simulink model "ellipsoidSMC"  (R2024a)
settings: Solver=ode45  StartTime=0  StopTime=350  FixedStep=0.01  MaxStep=0.01  RelTol=1e-4  AbsTol=1e-4  EnableMultiTasking=on
values from neighbouring files (symbols this model uses):
  simu = simulationClass()    [wecSimInputFile.m]
  waves = waveClass('regular')    [wecSimInputFile.m]
undefined symbols (not defined in the file or in its folder): body, controller, pto, X, Y, Z
libraries: nesl_utility x22, sm_lib x16, WECSim_Lib_Body_Elements x6, WECSim_Lib_Frames x1, vrlib x1, WECSim_Lib_PTOs x1
(part 2 of 3)

== system ellipsoidSMC/Rigid Body/Hydrodynamic Body/Structure ==
  note: Apply the total force to the body and calculate its response relative to the global reference frame.
      |
      | Output force to apply to another body.
  Total Force : Inport
  Body Properties : sm_lib/Body Elements/File Solid  ExtGeomFileName=geometry/elipsoid.stl  UnitType=Custom  ExtGeomFileUnits=m  StepReaderType=HEX  ExportConvexHullGeometry=off  InertiaType=Custom  BasedOnType=Density  Density=1000  DensityUnits=kg/(m^3)  Mass=body.mass  MassUnits=kg  CenterOfMass=[0 0 0]  CenterOfMassUnits=m  MomentsOfInertia=body.inertia  MomentsOfInertiaUnits=kg*m^2  ProductsOfInertia=body.inertiaProducts  ProductsOfInertiaUnits=kg*m^2  GraphicType=FromGeometry  MarkerShape=Sphere  MarkerSize=10  GraphicVisPropType=SimpleVisualProperties  GraphicDiffuseColor=body.viz.color  GraphicOpacity=body.viz.opacity  GraphicSpecularColor=[0.5 0.5 0.5 1.0]  GraphicAmbientColor=[0.15 0.15 0.15 1.0]  GraphicEmissiveColor=[0.0 0.0 0.0 1.0]  GraphicShininess=75  DoExposeReferenceFrame=on  SerializedFrames=<Frames/>
  External Force and Torque : sm_lib/Forces and Torques/External Force and Torque  EnableForceX=off  EnableForceY=off  EnableForceZ=off  EnableForce=on  ForceResolutionFrame=World  EnableTorqueX=off  EnableTorqueY=off  EnableTorqueZ=off  EnableTorque=on  TorqueResolutionFrame=World
  Motion Sensor : Subsystem
  Rigid Transform (Setup CG) : sm_lib/Frames and Transforms/Rigid Transform  RotationMethod=None  FollAlignAxisA=+X  BaseAlignAxisA=+Y  FollAlignAxisB=+Y  BaseAlignAxisB=+Z  RotationStandardAxis=+Y  RotationAngle=0.05  RotationAngleUnits=rad  RotationArbitraryAxis=[0.57735026918962584 0.57735026918962584 0.57735026918962584]  RotationSequenceAxes=FollowerAxes  RotationSequence=XYX  RotationSequenceAngles=[0 0 0]  RotationSequenceAnglesUnits=deg  RotationMatrix=[1 0 0; 0 1 0; 0 0 1]  Quaternion=[1 0 0 0]  TranslationMethod=Cartesian  TranslationCartesianOffset=body.centerGravity  TranslationCartesianOffsetUnits=m  TranslationStandardAxis=+Z  TranslationStandardOffset=0  TranslationStandardOffsetUnits=m  TranslationROffset=0  TranslationROffsetUnits=m  TranslationThetaOffset=0  TranslationThetaOffsetUnits=deg  TranslationZOffset=0  TranslationZOffsetUnits=m
  Rigid Transform (Setup Initial Disp) : sm_lib/Frames and Transforms/Rigid Transform  RotationMethod=ArbitraryAxis  FollAlignAxisA=+X  BaseAlignAxisA=+Y  FollAlignAxisB=+Y  BaseAlignAxisB=+Z  RotationStandardAxis=+Y  RotationAngle=body.initial.angle  RotationAngleUnits=rad  RotationArbitraryAxis=body.initial.axis  RotationSequenceAxes=FollowerAxes  RotationSequence=XYX  RotationSequenceAngles=[0 0 0]  RotationSequenceAnglesUnits=deg  RotationMatrix=[1 0 0; 0 1 0; 0 0 1]  Quaternion=[1 0 0 0]  TranslationMethod=Cartesian  TranslationCartesianOffset=body.initial.displacement  TranslationCartesianOffsetUnits=m  TranslationStandardAxis=+Z  TranslationStandardOffset=0  TranslationStandardOffsetUnits=m  TranslationROffset=0  TranslationROffsetUnits=m  TranslationThetaOffset=0  TranslationThetaOffsetUnits=deg  TranslationZOffset=0  TranslationZOffsetUnits=m
  Selector : Selector  InputPortWidth=6  IndexOptions=Index vector (dialog)  Indices=[1:3]  OutputSizes=1
  Selector1 : Selector  InputPortWidth=6  IndexOptions=Index vector (dialog)  Indices=[4:6]  OutputSizes=1
  Simulink-PS Converter1 : nesl_utility/Simulink-PS Converter  PhysicalDomain=network_engine_domain  SubClassName=ps_input  LeftPortType=input  RightPortType=output  PseudoPeriodic=off  Frequencies=[]  NoiseDistribution=none  NoiseParameters=[]  Unit=1  AffineConversion=off  FilteringAndDerivatives=zero  SimscapeFilterOrder=1  InputFilterTimeConstant=0.001  UdotUserProvided=1
  Simulink-PS Converter2 : nesl_utility/Simulink-PS Converter  PhysicalDomain=network_engine_domain  SubClassName=ps_input  LeftPortType=input  RightPortType=output  PseudoPeriodic=off  Frequencies=[]  NoiseDistribution=none  NoiseParameters=[]  Unit=1  AffineConversion=off  FilteringAndDerivatives=zero  SimscapeFilterOrder=1  InputFilterTimeConstant=0.001  UdotUserProvided=1
  World Frame : sm_lib/Frames and Transforms/World Frame
  Conn Free Surface : PMIOPort  Side=Right
  Response : Outport
  wires:
  Total Force/1 -> Selector1/1, Selector/1
  Selector/1 -> Simulink-PS Converter1/1
  Selector1/1 -> Simulink-PS Converter2/1
  Motion Sensor/1(Response) -> Response/1
  connections:
  External Force and Torque/LConn1 -- Simulink-PS Converter1/RConn1
  External Force and Torque/LConn2 -- Simulink-PS Converter2/RConn1
  Rigid Transform (Setup Initial Disp)/RConn1 -- Body Properties/RConn1 -- External Force and Torque/RConn1 -- Motion Sensor/RConn1
  Conn Free Surface/RConn1 -- Rigid Transform (Setup CG)/LConn1
  Rigid Transform (Setup Initial Disp)/LConn1 -- Rigid Transform (Setup CG)/RConn1
  World Frame/RConn1 -- Motion Sensor/LConn1

== system ellipsoidSMC/Rigid Body/Hydrodynamic Body/Wave Diffraction and Excitation Force Calculation ==
  note: The excitation force = F_wave * ramp function
  Time : Inport
  Displacement : Inport  Port=2
  WaveElv : Inport  Port=3
  Add : Sum
  Constant : Constant
  FexcInputs : Subsystem
  Less Than : RelationalOperator  Operator=<  OutDataTypeStr=boolean  RndMeth=Simplest  InputSameDT=off
  Linear Wave Excitation Force Variant Subsystem : Subsystem  Variant=on  VariantControl=sv_irregularWavesNonLinYaw_b1  mask{Nwave=waves(1)}
      mask prompts: Nwave "Wave Instance"
  Nonlinear FK Force Variant Subsystem : Subsystem  Variant=on
  Product : Product
  Ramp Function Time : Constant  Value=simu.rampTime
  Ramp function : Subsystem
  Switch : Switch  Criteria=u2 ~= 0  SaturateOnIntegerOverflow=off  InputSameDT=off
  F_Excitation : Outport  PortDimensions=body.dof
  wires:
  FexcInputs/3(Out3) -> Nonlinear FK Force Variant Subsystem/3(WaveElv)
  WaveElv/1 -> FexcInputs/3(WaveElv)
  Displacement/1 -> FexcInputs/2(Displacement)
  Time/1 -> FexcInputs/1(Time)
  FexcInputs/1(Out1) -> Nonlinear FK Force Variant Subsystem/1(Time), Linear Wave Excitation Force Variant Subsystem/1(Time), Ramp function/1(Time), Less Than/1
  FexcInputs/2(Out2) -> Nonlinear FK Force Variant Subsystem/2(Displacement), Linear Wave Excitation Force Variant Subsystem/2(Displacement)
  Constant/1 -> Switch/3
  Less Than/1 -> Switch/2
  Ramp function/1(R) -> Switch/1
  Ramp Function Time/1 -> Less Than/2
  Nonlinear FK Force Variant Subsystem/1(Nonlinear Excitation) -> Add/2
  Linear Wave Excitation Force Variant Subsystem/1(Linear Excitation) -> Add/1
  Product/1 -> F_Excitation/1  "F_Excitation"
  Add/1 -> Product/2  "F_wave"
  Switch/1 -> Product/1  "R"

== system ellipsoidSMC/Rigid Body/Hydrodynamic Body/Wave Radiation Forces Calculation ==
  note: F_AddedMass = AM * a
  Velocity : Inport
  Acceleration : Inport  Port=2
  Added Mass Matrix : Constant  Value=body.hydroForce.fAddedMass
  Product1 : Product  Multiplication=Matrix(*)
  SS CI and Constant-Damping-CoeVariant Subsystem : Subsystem  Variant=on
  F_RadiationDamping : Outport
  F_AddedMass : Outport  Port=2
  wires:
  Acceleration/1 -> Product1/2
  SS CI and Constant-Damping-CoeVariant Subsystem/1(Out1) -> F_RadiationDamping/1  "F_RadiationDamping"
  Velocity/1 -> SS CI and Constant-Damping-CoeVariant Subsystem/1(velocity)
  Product1/1 -> F_AddedMass/1  "F_AddedMass"
  Added Mass Matrix/1 -> Product1/1

== system ellipsoidSMC/Rigid Body/Hydrodynamic Body/Yaw Force Transforms ==
  F_Excitation : Inport
  F_RadiationDamping : Inport  Port=2
  In2 : Inport  Port=3
  F_AddedMass : Inport  Port=4
  F_Restoring : Inport  Port=5
  Constant : Constant  Value=body.yaw.option
  Yaw Force Transforms : MATLAB Function  TreatAsAtomicUnit=on
  Out1 : Outport
  Out2 : Outport  Port=2
  Out3 : Outport  Port=3
  Out4 : Outport  Port=4
  wires:
  Yaw Force Transforms/1(F_Excitation) -> Out1/1
  Yaw Force Transforms/3(F_AddedMass) -> Out3/1
  Yaw Force Transforms/2(F_RadiationDamping) -> Out2/1
  F_RadiationDamping/1 -> Yaw Force Transforms/2(dispGlobal)
  F_AddedMass/1 -> Yaw Force Transforms/4(F_AddedMassLocal)
  Yaw Force Transforms/4(F_Restoring) -> Out4/1
  F_Excitation/1 -> Yaw Force Transforms/5(F_ExcitationLocal)
  In2/1 -> Yaw Force Transforms/3(F_RadiationDampingLocal)
  F_Restoring/1 -> Yaw Force Transforms/6(F_RestoringLocal)
  Constant/1 -> Yaw Force Transforms/1(yaw)

== system ellipsoidSMC/Rigid Body/Hydrodynamic Body/Yaw Kinematic Transforms ==
  note: If simu.b2b == 0, no body to body interaction is used (noB2B)
      | If simu.b2b == 1, use body to body interaction (B2B)
  note: 1) Add Subsystem or Model blocks as valid variant choices.
      | 2) You cannot connect blocks at this level. At simulation, connectivity is automatically
      | determined, based on the active variant and port name matching.
  dispGlobal : Inport
  velGlobal : Inport  Port=2
  accGlobal : Inport  Port=3
  No B2B : Subsystem  VariantControl=sv_noB2B
  With B2B : Subsystem  VariantControl=sv_B2B
  dispLoc : Outport
  velLoc : Outport  Port=2
  accLoc : Outport  Port=3

== system ellipsoidSMC/Rigid Body/Non-Hydro Body/Structure ==
  note: Apply the total force to the body and calculate its response relative to the global reference frame.
      |
      | Output force to apply to another body.
  Total Force : Inport
  Body Properties : sm_lib/Body Elements/File Solid  ExtGeomFileName=geometry/elipsoid.stl  UnitType=Custom  ExtGeomFileUnits=m  StepReaderType=HEX  ExportConvexHullGeometry=off  InertiaType=Custom  BasedOnType=Density  Density=1000  DensityUnits=kg/(m^3)  Mass=body.mass  MassUnits=kg  CenterOfMass=[0 0 0]  CenterOfMassUnits=m  MomentsOfInertia=body.inertia  MomentsOfInertiaUnits=kg*m^2  ProductsOfInertia=body.inertiaProducts  ProductsOfInertiaUnits=kg*m^2  GraphicType=FromGeometry  MarkerShape=Sphere  MarkerSize=10  GraphicVisPropType=SimpleVisualProperties  GraphicDiffuseColor=body.viz.color  GraphicOpacity=body.viz.opacity  GraphicSpecularColor=[0.5 0.5 0.5 1.0]  GraphicAmbientColor=[0.15 0.15 0.15 1.0]  GraphicEmissiveColor=[0.0 0.0 0.0 1.0]  GraphicShininess=75  DoExposeReferenceFrame=on  SerializedFrames=<Frames/>
  External Force and Torque : sm_lib/Forces and Torques/External Force and Torque  EnableForceX=off  EnableForceY=off  EnableForceZ=off  EnableForce=on  ForceResolutionFrame=World  EnableTorqueX=off  EnableTorqueY=off  EnableTorqueZ=off  EnableTorque=on  TorqueResolutionFrame=World
  Motion Sensor : WECSim_Lib_Body_Elements/Rigid Body/Hydrodynamic Body/Structure/Motion Sensor  SystemSampleTime=-1  VariantActivationTime=update diagram  AllowFlexibleInterface=on  Latency=0  AutoFrameSizeCalculation=off
  Rigid Transform (Setup CG) : sm_lib/Frames and Transforms/Rigid Transform  RotationMethod=None  FollAlignAxisA=+X  BaseAlignAxisA=+Y  FollAlignAxisB=+Y  BaseAlignAxisB=+Z  RotationStandardAxis=+Y  RotationAngle=0.05  RotationAngleUnits=rad  RotationArbitraryAxis=[0.57735026918962584 0.57735026918962584 0.57735026918962584]  RotationSequenceAxes=FollowerAxes  RotationSequence=XYX  RotationSequenceAngles=[0 0 0]  RotationSequenceAnglesUnits=deg  RotationMatrix=[1 0 0; 0 1 0; 0 0 1]  Quaternion=[1 0 0 0]  TranslationMethod=Cartesian  TranslationCartesianOffset=body.centerGravity  TranslationCartesianOffsetUnits=m  TranslationStandardAxis=+Z  TranslationStandardOffset=0  TranslationStandardOffsetUnits=m  TranslationROffset=0  TranslationROffsetUnits=m  TranslationThetaOffset=0  TranslationThetaOffsetUnits=deg  TranslationZOffset=0  TranslationZOffsetUnits=m
  Rigid Transform (Setup Initial Disp) : sm_lib/Frames and Transforms/Rigid Transform  RotationMethod=ArbitraryAxis  FollAlignAxisA=+X  BaseAlignAxisA=+Y  FollAlignAxisB=+Y  BaseAlignAxisB=+Z  RotationStandardAxis=+Y  RotationAngle=body.initial.angle  RotationAngleUnits=rad  RotationArbitraryAxis=body.initial.axis  RotationSequenceAxes=FollowerAxes  RotationSequence=XYX  RotationSequenceAngles=[0 0 0]  RotationSequenceAnglesUnits=deg  RotationMatrix=[1 0 0; 0 1 0; 0 0 1]  Quaternion=[1 0 0 0]  TranslationMethod=Cartesian  TranslationCartesianOffset=body.initial.displacement  TranslationCartesianOffsetUnits=m  TranslationStandardAxis=+Z  TranslationStandardOffset=0  TranslationStandardOffsetUnits=m  TranslationROffset=0  TranslationROffsetUnits=m  TranslationThetaOffset=0  TranslationThetaOffsetUnits=deg  TranslationZOffset=0  TranslationZOffsetUnits=m
  Selector : Selector  InputPortWidth=6  IndexOptions=Index vector (dialog)  Indices=[1:3]  OutputSizes=1
  Selector1 : Selector  InputPortWidth=6  IndexOptions=Index vector (dialog)  Indices=[4:6]  OutputSizes=1
  Simulink-PS Converter1 : nesl_utility/Simulink-PS Converter  PhysicalDomain=network_engine_domain  SubClassName=ps_input  LeftPortType=input  RightPortType=output  PseudoPeriodic=off  Frequencies=[]  NoiseDistribution=none  NoiseParameters=[]  Unit=1  AffineConversion=off  FilteringAndDerivatives=zero  SimscapeFilterOrder=1  InputFilterTimeConstant=0.001  UdotUserProvided=1
  Simulink-PS Converter2 : nesl_utility/Simulink-PS Converter  PhysicalDomain=network_engine_domain  SubClassName=ps_input  LeftPortType=input  RightPortType=output  PseudoPeriodic=off  Frequencies=[]  NoiseDistribution=none  NoiseParameters=[]  Unit=1  AffineConversion=off  FilteringAndDerivatives=zero  SimscapeFilterOrder=1  InputFilterTimeConstant=0.001  UdotUserProvided=1
  World Frame : sm_lib/Frames and Transforms/World Frame
  Conn Free Surface : PMIOPort  Side=Right
  Response : Outport
  wires:
  Total Force/1 -> Selector1/1, Selector/1
  Selector/1 -> Simulink-PS Converter1/1
  Selector1/1 -> Simulink-PS Converter2/1
  Motion Sensor/1 -> Response/1
  connections:
  External Force and Torque/LConn1 -- Simulink-PS Converter1/RConn1
  External Force and Torque/LConn2 -- Simulink-PS Converter2/RConn1
  Motion Sensor/RConn1 -- Body Properties/RConn1 -- Rigid Transform (Setup Initial Disp)/RConn1 -- External Force and Torque/RConn1
  Conn Free Surface/RConn1 -- Rigid Transform (Setup CG)/LConn1
  Rigid Transform (Setup Initial Disp)/LConn1 -- Rigid Transform (Setup CG)/RConn1
  Motion Sensor/LConn1 -- World Frame/RConn1

== system ellipsoidSMC/Rigid Body/Hydrodynamic Body/B2B Subsystem/B2B ==
  CrossCoupling : Subsystem  mask{body=body}
      mask prompts: body "Body Number"
      mask help: This is used to
      mask init:
      | %In the initialization tab we place the code modifying the block
      | 
      | cb = gcb;
      | % position of initial blocks
      | set_param([cb '/vel1'],'Position',[200 1*50 240 (1*50+30)])
      | set_param([cb '/Mux1'], 'Position',[375 40 380 90])
      | set_param([cb '/vel'], 'Position',[410 59 440 71])
      | set_param([cb '/acc1'],'Position',[600 1*50 640 (1*50+30)])
      | set_param([cb '/Mux2'], 'Position',[775 40 780 90])
      | set_param([cb '/acc'], 'Position',[810 59 840 71])
      | set_param([cb '/Transport Delay1'], 'Position', [650 1*50 690 (1*50+30)])
      | 
      | % add/delete lines & blocks
      | newInputs = 0;
      | numbodies = body.total;
      | iBod = 2;
      | while iBod < 100
      |     try 
      |         find_system([cb,'/vel',num2str(iBod)],'Type','Block');
      |         if iBod > numbodies
      |             %delete 'From' blocks and lines if bodynumber > total bodies
      |             delete_line(cb,['vel',num2str(iBod),'/1'],['Mux',num2str(1),'/',num2str(iBod)])
      |             delete_line(cb,['acc',num2str(iBod),'/1'],['Transport Delay',num2str(iBod),'/1'])
      |             delete_line(cb,['Transport Delay',num2str(iBod),'/1'],['Mux',num2str(2),'/',num2str(iBod)])
      |             delete_block([cb '/vel',num2str(iBod)])
      |             delete_block([cb '/acc',num2str(iBod)])
      |             delete_block([cb '/Transport Delay',num2str(iBod)])
      |         end
      |     catch
      |         %set number of outputs for 'Mux Creator' blocks 
      |         if newInputs==0
      |             set_param([cb,'/Mux1'],'Inputs',num2str(numbodies))
      |             set_param([cb,'/Mux2'],'Inputs',num2str(numbodies))
      |         end
      |         if iBod <= numbodies
      |             newInputs = newInputs + 1;
      |             %add velocity 'From' block
      |             add_block('simulink/Signal Routing/From', [cb,'/vel',num2str(iBod)],'MakeNameUnique', 'on',...
      |             'Position',[200 iBod*50 240 (iBod*50+30)], 'BackgroundColor','green')
      |             h=[cb,'/vel',num2str(iBod)];
      |             responseName=['vel' num2str(iBod)];
      |             set_param(h,'GotoTag',responseName);
      |             %add acceleration 'From' block
      |             add_block('simulink/Signal Routing/From', [cb,'/acc',num2str(iBod)],'MakeNameUnique', 'on',...
      |             'Position',[600 iBod*50 640 (iBod*50+30)], 'BackgroundColor','green')
      |             h=[cb,'/acc',num2str(iBod)];
      |             responseName=['acc' num2str(iBod)];
      |             set_param(h,'GotoTag',responseName);
      |             % add transport delay block 
      |             add_block('simulink/Continuous/Transport Delay', [cb,'/Transport Delay',num2str(iBod)],'MakeNameUnique', 'on',...
      |             'Position',[650 iBod*50 690 (iBod*50+30)])
      |             h=[cb,'/Transport Delay',num2str(iBod)];
      |             set_param(h,'DelayTime',num2str(10e-8));
      |             %add lines
      |             add_line(cb,['vel',num2str(iBod),'/1'],['Mux',num2str(1),'/',num2str(iBod)])
      |             add_line(cb,['acc',num2str(iBod),'/1'],['Transport Delay',num2str(iBod),'/1'])
      |             add_line(cb,['Transport Delay',num2str(iBod),'/1'],['Mux',num2str(2),'/',num2str(iBod)])
      |             
      |         else
      |             break
      |         end
      |     end
      |     iBod = iBod + 1;
      | end
      mask Callback body: %customsat_callback('input',gcb)
      mask DialogControl DescGroupVar Prompt: Coupling Block
      mask DialogControl DescTextVar Prompt: This block transfers the velocity and acceleration vectors between bodies allowing for the coupled hydrodynamic forces to be calculated.  This block should not be included if there is only one body or if the hydrodynamic coupling parameter is set to 'No' in the rigid body block.
  vel : Outport
  acc : Outport  Port=2
  wires:
  CrossCoupling/2(acc) -> acc/1
  CrossCoupling/1(vel) -> vel/1

== system ellipsoidSMC/Rigid Body/Hydrodynamic Body/B2B Subsystem/noB2B ==
  vel_in : Inport
  acc_in : Inport  Port=2
  vel : Outport
  acc : Outport  Port=2
  wires:
  acc_in/1 -> acc/1
  vel_in/1 -> vel/1  "x"

== system ellipsoidSMC/Rigid Body/Hydrodynamic Body/Hydrostatic Restoring Force Calculation/Linear and Nonlinear Restoring Force Variant Subsystem ==
  note: 1) Add Subsystem or Model blocks as valid variant choices.
      | 2) You cannot connect blocks at this level. At simulation, connectivity is automatically
      | determined, based on the active variant and port name matching.
  note: If simu.nlHydro == 0, use the linear force option.
      | If simu.nlHydro > 0, use the nonlinear force option.
  In1 : Inport
  In2 : Inport  Port=2
  Linear Hydrostatic Restoring Force : Subsystem  VariantControl=sv_b1_linearHydro
  Nonlinear Hydrostatic Restoring Force : Subsystem  VariantControl=sv_b1_nonlinearHydro
  Out1 : Outport

== system ellipsoidSMC/Rigid Body/Hydrodynamic Body/Morison Element and Viscous Damping Force Calculation/Morison Element Variant Subsystem ==
  note: 1) Add Subsystem or Model blocks as valid variant choices.
      | 2) You cannot connect blocks at this level. At simulation, connectivity is automatically
      | determined, based on the active variant and port name matching.
  note: If body.morisonElement.option == 0, Morison element is off and the Morison force is 0
      | If body.morisonElement.option == 1 | 2, Morison element is on
  displacement : Inport
  velocity : Inport  Port=2
  acceleration : Inport  Port=3
  time : Inport  Port=4
  Morison Element Off : Subsystem  VariantControl=sv_b1_MEOff
  Morison Element On : Subsystem  Variant=on  VariantControl=sv_b1_MEOn
  morison_force : Outport

== system ellipsoidSMC/Rigid Body/Hydrodynamic Body/Nonlinear Wave Elevation/Linear or Instantaneous Free Surface ==
  note: 1) Add Subsystem or Model blocks as valid variant choices.
      | 2) You cannot connect blocks at this level. At simulation, connectivity is automatically
      | determined, based on the active variant and port name matching.
  note: If simu.nlHydro < 2, use the mean water free surface.
      | If simu.nlHydro == 2, use the instantaneous water free surface
  In1 : Inport
  In2 : Inport  Port=2
  Instantaneous Water Free Surface : Subsystem  VariantControl=sv_b1_instFS
  Mean Water Free Surface : Subsystem  VariantControl=sv_b1_meanFS
  Out1 : Outport

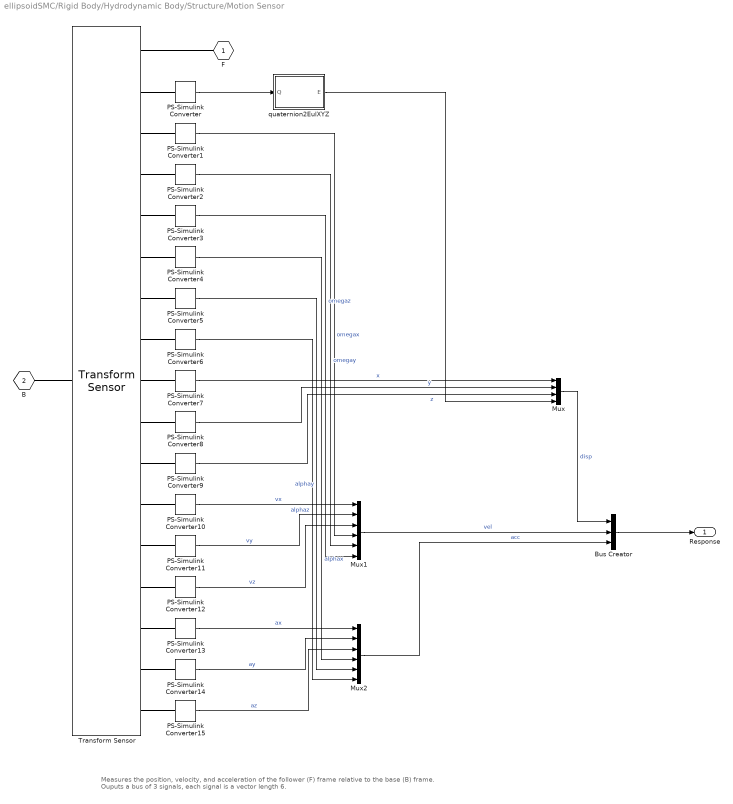
== system ellipsoidSMC/Rigid Body/Hydrodynamic Body/Structure/Motion Sensor ==
  note: Measures the position, velocity, and acceleration of the follower (F) frame relative to the base (B) frame.
      | Ouputs a bus of 3 signals, each signal is a vector length 6.
  Bus Creator : BusCreator  Inputs=3
  Mux : Mux
  Mux1 : Mux  Inputs=6
  Mux2 : Mux  Inputs=6
  PS-Simulink Converter{,1..15} (16 alike) : nesl_utility/PS-Simulink Converter  PhysicalDomain=network_engine_domain  SubClassName=ps_output  LeftPortType=input  RightPortType=output  PseudoPeriodic=off  Frequencies=[]  VectorFormat=1-D array  Unit=1  AffineConversion=off
  Transform Sensor : sm_lib/Frames and Transforms/Transform Sensor  MeasurementFrame=World  RotationSequence=XYX  SenseAngle=off  SenseAxis=off  SenseQ=on  SenseR=off  SenseRotationSequence=off  SenseOmegaX=on  SenseOmegaY=on  SenseOmegaZ=on  SenseOmega=off  SenseQDot=off  SenseRDot=off  SenseRotationSequenceDot=off  SenseAlphaX=on  SenseAlphaY=on  SenseAlphaZ=on  SenseAlpha=off  SenseQDDot=off  SenseRDDot=off  SenseX=on  SenseY=on  SenseZ=on  SenseXYZ=off  SenseRad=off  SenseAzim=off  SenseDist=off  SenseInc=off  SenseXDot=on  SenseYDot=on  SenseZDot=on  SenseXYZDot=off  SenseRadDot=off  SenseAzimDot=off  SenseDistDot=off  SenseIncDot=off  SenseXDDot=on  SenseYDDot=on  SenseZDDot=on  SenseXYZDDot=off  SenseRadDDot=off  SenseAzimDDot=off  SenseDistDDot=off  SenseIncDDot=off
  quaternion2EulXYZ : MATLAB Function  TreatAsAtomicUnit=on
  F : PMIOPort  Side=Right
  B : PMIOPort  Port=2  Side=Left
  Response : Outport
  wires:
  PS-Simulink Converter/1 -> quaternion2EulXYZ/1(Q)
  quaternion2EulXYZ/1(E) -> Mux/4
  PS-Simulink Converter4/1 -> Mux2/4  "alphax"
  PS-Simulink Converter10/1 -> Mux1/1  "vx"
  PS-Simulink Converter12/1 -> Mux1/3  "vz"
  PS-Simulink Converter13/1 -> Mux2/1  "ax"
  PS-Simulink Converter14/1 -> Mux2/2  "ay"
  Mux/1 -> Bus Creator/1  "disp"
  Mux1/1 -> Bus Creator/2  "vel"
  Mux2/1 -> Bus Creator/3  "acc"
  PS-Simulink Converter7/1 -> Mux/1  "x"
  PS-Simulink Converter8/1 -> Mux/2  "y"
  PS-Simulink Converter9/1 -> Mux/3  "z"
  PS-Simulink Converter5/1 -> Mux2/5  "alphay"
  PS-Simulink Converter6/1 -> Mux2/6  "alphaz"
  PS-Simulink Converter1/1 -> Mux1/4  "omegax"
  PS-Simulink Converter2/1 -> Mux1/5  "omegay"
  PS-Simulink Converter11/1 -> Mux1/2  "vy"
  PS-Simulink Converter3/1 -> Mux1/6  "omegaz"
  PS-Simulink Converter15/1 -> Mux2/3  "az"
  Bus Creator/1 -> Response/1
  connections:
  Transform Sensor/RConn16 -- PS-Simulink Converter14/LConn1
  PS-Simulink Converter13/LConn1 -- Transform Sensor/RConn15
  PS-Simulink Converter12/LConn1 -- Transform Sensor/RConn14
  Transform Sensor/RConn13 -- PS-Simulink Converter11/LConn1
  PS-Simulink Converter10/LConn1 -- Transform Sensor/RConn12
  PS-Simulink Converter9/LConn1 -- Transform Sensor/RConn11
  Transform Sensor/RConn10 -- PS-Simulink Converter8/LConn1
  PS-Simulink Converter7/LConn1 -- Transform Sensor/RConn9
  Transform Sensor/RConn8 -- PS-Simulink Converter6/LConn1
  PS-Simulink Converter5/LConn1 -- Transform Sensor/RConn7
  Transform Sensor/RConn6 -- PS-Simulink Converter4/LConn1
  PS-Simulink Converter3/LConn1 -- Transform Sensor/RConn5
  Transform Sensor/RConn4 -- PS-Simulink Converter2/LConn1
  PS-Simulink Converter1/LConn1 -- Transform Sensor/RConn3
  Transform Sensor/RConn2 -- PS-Simulink Converter/LConn1
  PS-Simulink Converter15/LConn1 -- Transform Sensor/RConn17
  Transform Sensor/RConn1 -- F/RConn1
  B/RConn1 -- Transform Sensor/LConn1

== system ellipsoidSMC/Rigid Body/Hydrodynamic Body/Wave Diffraction and Excitation Force Calculation/FexcInputs ==
  Time : Inport
  Displacement : Inport  Port=2
  WaveElv : Inport  Port=3
  Out1 : Outport
  Out2 : Outport  Port=2
  Out3 : Outport  Port=3
  wires:
  Displacement/1 -> Out2/1
  Time/1 -> Out1/1
  WaveElv/1 -> Out3/1

== system ellipsoidSMC/Rigid Body/Hydrodynamic Body/Wave Diffraction and Excitation Force Calculation/Linear Wave Excitation Force Variant Subsystem ==
  note: 1) Add Subsystem or Model blocks as valid variant choices.
      | 2) You cannot connect blocks at this level. At simulation, connectivity is automatically
      | determined, based on the active variant and port name matching.
  note: No wave includes wave.type == 'noWave' or 'noWaveCIC'
      | Regular wave includes wave.type == 'regular' or 'regularCIC'
      | Irregular wave includes wave.type == 'irregular' or 'spectrumImport'
  Time : Inport
  Displacement : Inport  Port=2
  Irregular Wave Excitation Force : Subsystem  VariantControl=sv_irregularWaves_b1
  Irregular Wave NonLinearYaw : Subsystem  VariantControl=sv_irregularWavesYaw_b1
  No Wave Excitation Force : Subsystem  VariantControl=sv_noWave
  Regular Wave Excitation Force : Subsystem  VariantControl=sv_regularWaves_b1
  Regular Wave NonLinear Yaw : Subsystem  VariantControl=sv_regularWavesYaw_b1
  User Defined Wave Excitation Force : Subsystem  VariantControl=sv_udfWaves
  Linear Excitation : Outport

== system ellipsoidSMC/Rigid Body/Hydrodynamic Body/Wave Diffraction and Excitation Force Calculation/Nonlinear FK Force Variant Subsystem ==
  note: 1) Add Subsystem or Model blocks as valid variant choices.
      | 2) You cannot connect blocks at this level. At simulation, connectivity is automatically
      | determined, based on the active variant and port name matching.
  note: If simu.nlHydro == 0, use No Nonlinear FroudeKrylov force option (nonlinear force is zero),
      | If simu.nlHydro > 0, use the Nonlinear FroudeKrylov force option,
  Time : Inport
  Displacement : Inport  Port=2
  WaveElv : Inport  Port=3
  No Nonlinear FroudeKrylov Force : Subsystem  VariantControl=sv_b1_linearHydro
  With Nonlinear FroudeKrylov Force : Subsystem  TreatAsAtomicUnit=on  SystemSampleTime=simu.nonlinearDt  VariantControl=sv_b1_nonlinearHydro
  Nonlinear Excitation : Outport

== system ellipsoidSMC/Rigid Body/Hydrodynamic Body/Wave Diffraction and Excitation Force Calculation/Ramp function ==
  note: The ramp function R, is a smooth function:
      | R = (sin(3*pi/2 + pi * t/Tr) + 1)/2 from t=0 to t=Tr
  Time : Inport
  Add1 : Sum
  Add2 : Sum
  Constant1 : Constant  Value=1/2
  Constant2 : Constant
  Constant3 : Constant  Value=3*pi/2
  Constant4 : Constant  Value=pi
  Divide : Product  Inputs=*/
  Product1 : Product
  Product2 : Product
  Ramp Time : Constant  Value=simu.rampTime
  Sine Wave Function : Sin  TimeSource=Use external signal  SampleTime=0
  R : Outport
  wires:
  Product1/1 -> R/1
  Constant2/1 -> Add1/1
  Constant3/1 -> Add2/2  "phase"
  Ramp Time/1 -> Divide/2  "t_ramp"
  Divide/1 -> Product2/2  "frequency"
  Add1/1 -> Product1/1
  Constant4/1 -> Divide/1
  Add2/1 -> Sine Wave Function/1
  Product2/1 -> Add2/1
  Time/1 -> Product2/1
  Sine Wave Function/1 -> Add1/2
  Constant1/1 -> Product1/2

== system ellipsoidSMC/Rigid Body/Hydrodynamic Body/Wave Radiation Forces Calculation/SS CI and Constant-Damping-CoeVariant Subsystem ==
  note: 1) Add Subsystem or Model blocks as valid variant choices.
      | 2) You cannot connect blocks at this level. At simulation, connectivity is automatically
      | determined, based on the active variant and port name matching.
  note: If the wave type is 'noWave' or 'regular' use constant coefficients.
      | If another wave type and simu.Calc ~= 1, use convolution integral calculation
      | If another wave type and simu.Calc == 1, use the state space calculation
      | If another wave type and simu.FIR == 1, use the FIR filter calculation
  velocity : Inport
  Constant Coefficients : Subsystem  VariantControl=sv_constantCoeff
  Convolution Integral Calculation : Subsystem  VariantControl=sv_convolution
  FIR Filter Calculation : Subsystem  VariantControl=sv_FIR
  "State-Space Calculation " : Subsystem  VariantControl=sv_stateSpace
  Out1 : Outport

== system ellipsoidSMC/Rigid Body/Hydrodynamic Body/Yaw Kinematic Transforms/No B2B ==
  note: If body.yaw.option == 1, interpolate the BEM coefficients to account for the effective change in the incoming wave direction.
  dispGlobal : Inport
  velGlobal : Inport  Port=2
  accGlobal : Inport  Port=3
  Constant : Constant  Value=body.yaw.option
  Yaw Kinematic Transforms : MATLAB Function  TreatAsAtomicUnit=on
  dispLoc : Outport
  velLoc : Outport  Port=2
  accLoc : Outport  Port=3
  wires:
  Yaw Kinematic Transforms/3(accLoc) -> accLoc/1
  Yaw Kinematic Transforms/1(dispLoc) -> dispLoc/1
  Yaw Kinematic Transforms/2(velLoc) -> velLoc/1
  Constant/1 -> Yaw Kinematic Transforms/1(yaw)
  accGlobal/1 -> Yaw Kinematic Transforms/4(accGlobal)
  velGlobal/1 -> Yaw Kinematic Transforms/3(velGlobal)
  dispGlobal/1 -> Yaw Kinematic Transforms/2(dispGlobal)

== system ellipsoidSMC/Rigid Body/Hydrodynamic Body/Yaw Kinematic Transforms/With B2B ==
  note: If body.yaw.option == 1, interpolate the BEM coefficients to account for the effective change in the incoming wave direction.
  dispGlobal : Inport
  velGlobal : Inport  Port=2
  accGlobal : Inport  Port=3
  Constant : Constant  Value=body.yaw.option
  Yaw Kinematic Transforms : MATLAB Function  TreatAsAtomicUnit=on
  dispLoc : Outport
  velLoc : Outport  Port=2
  accLoc : Outport  Port=3
  wires:
  accGlobal/1 -> Yaw Kinematic Transforms/4(accGlobal)
  velGlobal/1 -> Yaw Kinematic Transforms/3(velGlobal)
  dispGlobal/1 -> Yaw Kinematic Transforms/2(dispGlobal)
  Yaw Kinematic Transforms/3(accLoc) -> accLoc/1
  Yaw Kinematic Transforms/2(velLoc) -> velLoc/1
  Yaw Kinematic Transforms/1(dispLoc) -> dispLoc/1
  Constant/1 -> Yaw Kinematic Transforms/1(yaw)

== system ellipsoidSMC/Rigid Body/Hydrodynamic Body/B2B Subsystem/B2B/CrossCoupling ==
  note: CrossCoupling block is updated by its mask initialization, which is only called on when a simulation is run. 'From' blocks are automatically created and connected based on the number of bodies in the simulation.
  Mux1 : Mux  Inputs=2
  Mux2 : Mux  Inputs=2
  Transport Delay1 : TransportDelay  DelayTime=10e-8
  Transport Delay2 : TransportDelay  DelayTime=1e-07
  vel : Outport
  acc : Outport  Port=2
  wires:
  Transport Delay2/1 -> Mux2/2
  [acc2] -> Transport Delay2/1
  [vel2] -> Mux1/2
  Transport Delay1/1 -> Mux2/1
  Mux2/1 -> acc/1
  [acc1] -> Transport Delay1/1
  Mux1/1 -> vel/1
  [vel1] -> Mux1/1

== system ellipsoidSMC/Rigid Body/Hydrodynamic Body/Hydrostatic Restoring Force Calculation/Linear and Nonlinear Restoring Force Variant Subsystem/Linear Hydrostatic Restoring Force ==
  note: The total hydrostatic restoring force is due to a linear stiffness, the vertical buoyancy force (gravity - buoyancy) and a rotational buoyancy force if the center of gravity is not aligned with the center of buoyancy.
      |
      | F_restoring = F_linearRestoringStiffness + F_NetBuoyancy
      |
      | F_linear restoring = hydrostatic restoring coefficient * displacement
      | F_NetBuoyancy = F_gravity - F_buoyancy + F_rotational_buoyancy
      |
      | F_rotational_buoyancy = (cb-cg) x F_buoyancy
      | F_buoyancy = rho*g*V_0
      | F_gravity = m*g
  In1 : Inport
  Add : Sum
  Body Mass : Constant  Value=body.hydroForce.storage.mass
  Linear Restoring Coefficient Matrix : Constant  Value=body.hydroForce.linearHydroRestCoef
  Net Buoyancy Force : Subsystem
  Product2 : Product  Multiplication=Matrix(*)
  Out1 : Outport
  wires:
  Body Mass/1 -> Net Buoyancy Force/1(Body Mass)  "m"
  Net Buoyancy Force/1(F_NetBuoyancy) -> Add/1  "Net buoyancy force"
  Product2/1 -> Add/2  "Linear Restoring Force"
  Add/1 -> Out1/1  "F_Restoring"
  Linear Restoring Coefficient Matrix/1 -> Product2/1  "K"
  In1/1 -> Product2/2  "x"

== system ellipsoidSMC/Rigid Body/Hydrodynamic Body/Hydrostatic Restoring Force Calculation/Linear and Nonlinear Restoring Force Variant Subsystem/Nonlinear Hydrostatic Restoring Force ==
  In1 : Inport
  In2 : Inport  Port=2
  Body Mass2 : Constant  Value=body.hydroForce.storage.mass
  Center of Gravity : Constant  Value=body.centerGravity
  Gravity2 : Constant  Value=simu.gravity
  Rate Transition : RateTransition
  Rate Transition1 : RateTransition
  Restoring Forces : MATLAB Function  TreatAsAtomicUnit=on  SystemSampleTime=simu.nonlinearDt
  STL areas : Constant  Value=body.geometry.area
  STL centers : Constant  Value=body.geometry.center
  STL normal vectors : Constant  Value=body.geometry.norm
  To Workspace1 : ToWorkspace  VariableName=body1_hspressure_out  SaveFormat=Structure With Time  SampleTime=-1
      settings: Decimation=round(simu.dtOut/simu.dt,0)
  Water Density1 : Constant  Value=simu.rho
  Out1 : Outport
  wires:
  Rate Transition/1 -> Out1/1
  Restoring Forces/1(f) -> Rate Transition/1
  Rate Transition1/1 -> To Workspace1/1
  Restoring Forces/2(p) -> Rate Transition1/1
  Body Mass2/1 -> Restoring Forces/9(mass)
  STL areas/1 -> Restoring Forces/5(area)
  In2/1 -> Restoring Forces/2(elv)
  STL centers/1 -> Restoring Forces/3(center)
  STL normal vectors/1 -> Restoring Forces/4(tnorm)
  Water Density1/1 -> Restoring Forces/6(rho)
  Gravity2/1 -> Restoring Forces/7(g)  "g"
  Center of Gravity/1 -> Restoring Forces/8(cg)
  In1/1 -> Restoring Forces/1(x)

== system ellipsoidSMC/Rigid Body/Hydrodynamic Body/Morison Element and Viscous Damping Force Calculation/Morison Element Variant Subsystem/Morison Element Off ==
  Constant : Constant  Value=zeros(1,body.dof)
  morison_force : Outport
  wires:
  Constant/1 -> morison_force/1

== system ellipsoidSMC/Rigid Body/Hydrodynamic Body/Morison Element and Viscous Damping Force Calculation/Morison Element Variant Subsystem/Morison Element On ==
  note: 1) Add Subsystem or Model blocks as valid variant choices.
      | 2) You cannot connect blocks at this level. At simulation, connectivity is automatically
      | determined, based on the active variant and port name matching.
  note: Chooses the appropriate Morison element variant dependent on the wave type. Note that if passive yaw is used, no block is chosen.
      |
      | If wave.type == 'noWave' | 'noWaveCIC' use No Wave Morison element
      | If wave.type == 'regularWave' | 'regularWaveCIC' use Regular Wave Morison element
      | If wave.type == 'irregularWave' or 'spectrumImport' use Irregular Wave Morison element
  displacement : Inport
  velocity : Inport  Port=2
  acceleration : Inport  Port=3
  time : Inport  Port=4
  Irregular Wave Morison Force : Subsystem  TreatAsAtomicUnit=on  SystemSampleTime=simu.morisonDt  VariantControl=sv_irregularWaves_b1
  No Wave Morison Force : Subsystem  VariantControl=sv_noWave
  Regular Wave Morison Force : Subsystem  TreatAsAtomicUnit=on  SystemSampleTime=simu.morisonDt  VariantControl=sv_regularWaves_b1
  morison_force : Outport

== system ellipsoidSMC/Rigid Body/Hydrodynamic Body/Nonlinear Wave Elevation/Linear or Instantaneous Free Surface/Instantaneous Water Free Surface ==
  note: Calculate the instantaneous wave elevation for the nonlinear hydrodynamics options.
  In1 : Inport
  In2 : Inport  Port=2
  Center of Gravity : Constant  Value=body.centerGravity
  Frequency Spacing : Constant  Value=waves.dOmega
  Instantaneous FS : MATLAB Function  TreatAsAtomicUnit=on
  Ramp Time : Constant  Value=simu.rampTime
  STL Centers : Constant  Value=body.geometry.center
  Wave Amplitude : Constant  Value=waves.amplitude
  Wave Direction : Constant  Value=waves.direction
  Wave Frequency : Constant  Value=waves.omega
  Wave Number : Constant  Value=waves.wavenumber
  Wave Random Phase : Constant  Value=waves.phase
  Wave Type Number : Constant  Value=waves.typeNum
  Out1 : Outport
  wires:
  Wave Amplitude/1 -> Instantaneous FS/4(AH)
  Wave Direction/1 -> Instantaneous FS/12(waveDir)
  In1/1 -> Instantaneous FS/1(x)
  In2/1 -> Instantaneous FS/9(t)
  Frequency Spacing/1 -> Instantaneous FS/6(dw)
  Wave Random Phase/1 -> Instantaneous FS/11(phaseRand)
  Ramp Time/1 -> Instantaneous FS/10(rampT)
  Wave Type Number/1 -> Instantaneous FS/8(typeNum)
  Wave Frequency/1 -> Instantaneous FS/5(w)
  Wave Number/1 -> Instantaneous FS/7(k)
  Center of Gravity/1 -> Instantaneous FS/3(cg)
  STL Centers/1 -> Instantaneous FS/2(center)
  Instantaneous FS/1(f) -> Out1/1

== system ellipsoidSMC/Rigid Body/Hydrodynamic Body/Nonlinear Wave Elevation/Linear or Instantaneous Free Surface/Mean Water Free Surface ==
  note: The mean water surface is always zero.
  zero : Constant  Value=0
  Out1 : Outport
  wires:
  zero/1 -> Out1/1

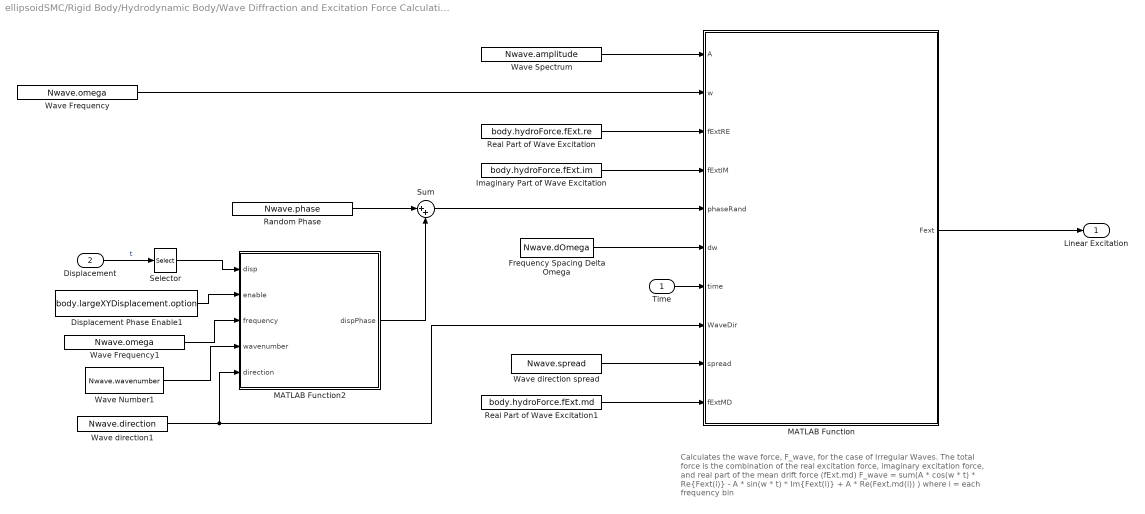
== system ellipsoidSMC/Rigid Body/Hydrodynamic Body/Wave Diffraction and Excitation Force Calculation/Linear Wave Excitation Force Variant Subsystem/Irregular Wave Excitation Force ==
  note: Calculates the wave force, F_wave, for the case of Irregular Waves.
      |
      | The total force is the combination of the real excitation force, imaginary excitation force, and real part of the mean drift force (fExt.md)
      |
      | F_wave =   sum(A * cos(w * t) * Re{Fext(i)}
      |                            -  A * sin(w * t) * Im{Fext(i)}
      |                            + A * Re(Fext.md(i))
      |                            )
      |
      | where i = each frequency bin
  Time : Inport
  Displacement : Inport  Port=2
  Displacement Phase Enable1 : Constant  Value=body.largeXYDisplacement.option
  Frequency Spacing Delta Omega : Constant  Value=Nwave.dOmega  VectorParams1D=off
  Imaginary Part of Wave Excitation : Constant  Value=body.hydroForce.fExt.im  VectorParams1D=off
  MATLAB Function : MATLAB Function  TreatAsAtomicUnit=on
  MATLAB Function2 : MATLAB Function  TreatAsAtomicUnit=on
  Random Phase : Constant  Value=Nwave.phase  VectorParams1D=off
  Real Part of Wave Excitation : Constant  Value=body.hydroForce.fExt.re  VectorParams1D=off
  Real Part of Wave Excitation1 : Constant  Value=body.hydroForce.fExt.md  VectorParams1D=off
  Selector : Selector  IndexOptions=Index vector (dialog)  Indices=[1 2]  OutputSizes=1
  Sum : Sum  Inputs=|++
  Wave Frequency : Constant  Value=Nwave.omega  VectorParams1D=off
  Wave Frequency1 : Constant  Value=Nwave.omega  VectorParams1D=off
  Wave Number1 : Constant  Value=Nwave.wavenumber
  Wave Spectrum : Constant  Value=Nwave.amplitude  VectorParams1D=off
  Wave direction spread : Constant  Value=Nwave.spread  VectorParams1D=off
  Wave direction1 : Constant  Value=Nwave.direction  VectorParams1D=off
  Linear Excitation : Outport
  wires:
  Wave direction1/1 -> MATLAB Function2/5(direction), MATLAB Function/8(WaveDir)
  Wave Number1/1 -> MATLAB Function2/4(wavenumber)
  Displacement/1 -> Selector/1  "t"
  Selector/1 -> MATLAB Function2/1(disp)
  Displacement Phase Enable1/1 -> MATLAB Function2/2(enable)
  Wave Frequency1/1 -> MATLAB Function2/3(frequency)
  Random Phase/1 -> Sum/1
  Sum/1 -> MATLAB Function/5(phaseRand)
  MATLAB Function2/1(dispPhase) -> Sum/2
  Real Part of Wave Excitation1/1 -> MATLAB Function/10(fExtMD)
  Wave direction spread/1 -> MATLAB Function/9(spread)
  Frequency Spacing Delta Omega/1 -> MATLAB Function/6(dw)
  Time/1 -> MATLAB Function/7(time)
  Wave Spectrum/1 -> MATLAB Function/1(A)
  Real Part of Wave Excitation/1 -> MATLAB Function/3(fExtRE)
  Imaginary Part of Wave Excitation/1 -> MATLAB Function/4(fExtIM)
  Wave Frequency/1 -> MATLAB Function/2(w)
  MATLAB Function/1(Fext) -> Linear Excitation/1

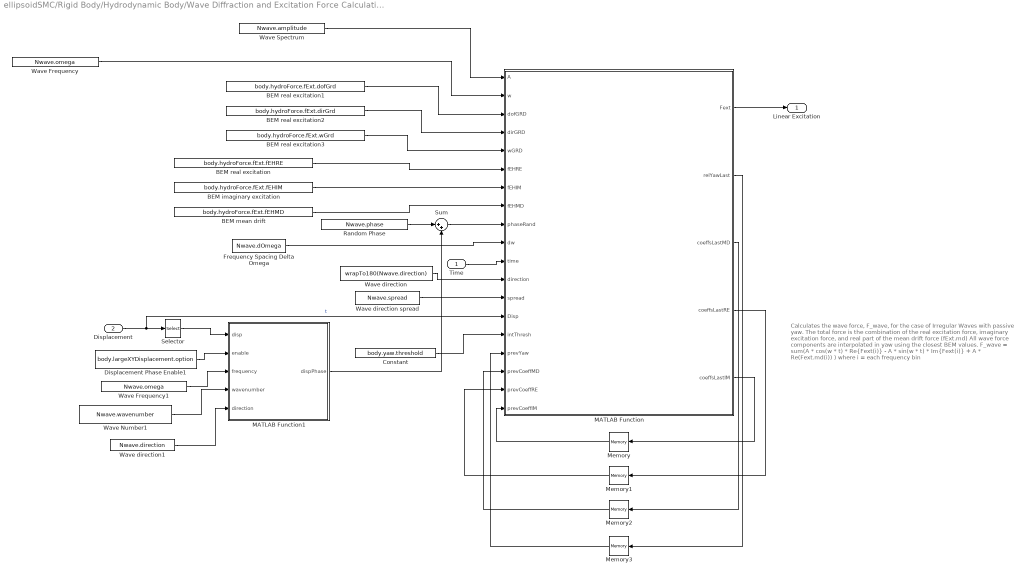
== system ellipsoidSMC/Rigid Body/Hydrodynamic Body/Wave Diffraction and Excitation Force Calculation/Linear Wave Excitation Force Variant Subsystem/Irregular Wave NonLinearYaw ==
  note: Calculates the wave force, F_wave, for the case of Irregular Waves with passive yaw.
      |
      | The total force is the combination of the real excitation force, imaginary excitation force, and real part of the mean drift force (fExt.md)
      |
      | All wave force components are interpolated in yaw using the closest BEM values.
      |
      | F_wave =   sum(A * cos(w * t) * Re{Fext(i)}
      |                            -  A * sin(w * t) * Im{Fext(i)}
      |                            + A * Re(Fext.md(i))
      |                            )
      |
      | where i = each frequency bin
  Time : Inport
  Displacement : Inport  Port=2
  BEM imaginary excitation : Constant  Value=body.hydroForce.fExt.fEHIM  VectorParams1D=off
  BEM mean drift : Constant  Value=body.hydroForce.fExt.fEHMD  VectorParams1D=off
  BEM real excitation : Constant  Value=body.hydroForce.fExt.fEHRE  VectorParams1D=off
  BEM real excitation1 : Constant  Value=body.hydroForce.fExt.dofGrd  VectorParams1D=off
  BEM real excitation2 : Constant  Value=body.hydroForce.fExt.dirGrd  VectorParams1D=off
  BEM real excitation3 : Constant  Value=body.hydroForce.fExt.wGrd  VectorParams1D=off
  Constant : Constant  Value=body.yaw.threshold
  Displacement Phase Enable1 : Constant  Value=body.largeXYDisplacement.option
  Frequency Spacing Delta Omega : Constant  Value=Nwave.dOmega  VectorParams1D=off
  MATLAB Function : MATLAB Function  TreatAsAtomicUnit=on
  MATLAB Function1 : MATLAB Function  TreatAsAtomicUnit=on
  Memory{,1..3} (4 alike) : Memory  InheritSampleTime=on  LinearizeAsDelay=on
  Random Phase : Constant  Value=Nwave.phase  VectorParams1D=off
  Selector : Selector  IndexOptions=Index vector (dialog)  Indices=[1 2]  OutputSizes=1
  Sum : Sum  Inputs=|++
  Wave Frequency : Constant  Value=Nwave.omega  VectorParams1D=off
  Wave Frequency1 : Constant  Value=Nwave.omega  VectorParams1D=off
  Wave Number1 : Constant  Value=Nwave.wavenumber
  Wave Spectrum : Constant  Value=Nwave.amplitude  VectorParams1D=off
  Wave direction : Constant  Value=wrapTo180(Nwave.direction)  VectorParams1D=off
  Wave direction spread : Constant  Value=Nwave.spread  VectorParams1D=off
  Wave direction1 : Constant  Value=Nwave.direction  VectorParams1D=off
  Linear Excitation : Outport
  wires:
  MATLAB Function1/1(dispPhase) -> Sum/2
  Wave direction1/1 -> MATLAB Function1/5(direction)
  Wave Number1/1 -> MATLAB Function1/4(wavenumber)
  Displacement/1 -> Selector/1, MATLAB Function/14(Disp)  "t"
  Selector/1 -> MATLAB Function1/1(disp)
  Displacement Phase Enable1/1 -> MATLAB Function1/2(enable)
  Wave Frequency1/1 -> MATLAB Function1/3(frequency)
  Sum/1 -> MATLAB Function/9(phaseRand)
  Random Phase/1 -> Sum/1
  Time/1 -> MATLAB Function/11(time)
  Wave direction spread/1 -> MATLAB Function/13(spread)
  BEM mean drift/1 -> MATLAB Function/8(fEHMD)
  Wave Spectrum/1 -> MATLAB Function/1(A)
  BEM real excitation1/1 -> MATLAB Function/3(dofGRD)
  Wave Frequency/1 -> MATLAB Function/2(w)
  Memory/1 -> MATLAB Function/19(prevCoeffIM)
  BEM real excitation/1 -> MATLAB Function/6(fEHRE)
  MATLAB Function/3(coeffsLastMD) -> Memory2/1
  Constant/1 -> MATLAB Function/15(intThresh)
  BEM imaginary excitation/1 -> MATLAB Function/7(fEHIM)
  Memory3/1 -> MATLAB Function/16(prevYaw)
  MATLAB Function/5(coeffsLastIM) -> Memory/1
  Wave direction/1 -> MATLAB Function/12(direction)
  Frequency Spacing Delta Omega/1 -> MATLAB Function/10(dw)
  BEM real excitation2/1 -> MATLAB Function/4(dirGRD)
  BEM real excitation3/1 -> MATLAB Function/5(wGRD)
  Memory2/1 -> MATLAB Function/17(prevCoeffMD)
  MATLAB Function/2(relYawLast) -> Memory3/1
  MATLAB Function/4(coeffsLastRE) -> Memory1/1
  Memory1/1 -> MATLAB Function/18(prevCoeffRE)
  MATLAB Function/1(Fext) -> Linear Excitation/1

== system ellipsoidSMC/Rigid Body/Hydrodynamic Body/Wave Diffraction and Excitation Force Calculation/Linear Wave Excitation Force Variant Subsystem/No Wave Excitation Force ==
  Constant : Constant  Value=zeros(1,body.dof)
  Linear Excitation : Outport
  wires:
  Constant/1 -> Linear Excitation/1

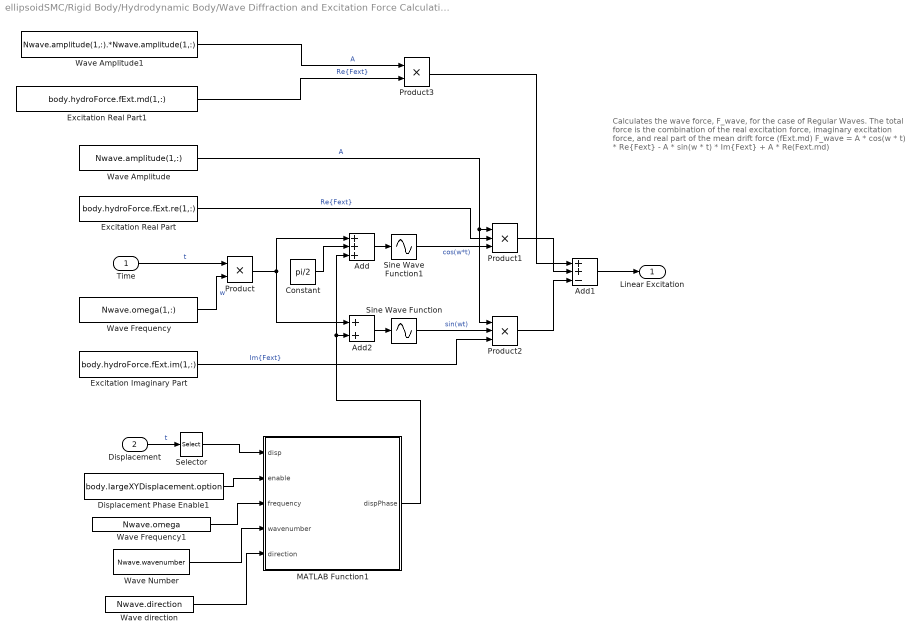
== system ellipsoidSMC/Rigid Body/Hydrodynamic Body/Wave Diffraction and Excitation Force Calculation/Linear Wave Excitation Force Variant Subsystem/Regular Wave Excitation Force ==
  note: Calculates the wave force, F_wave, for the case of Regular Waves.
      |
      | The total force is the combination of the real excitation force, imaginary excitation force, and real part of the mean drift force (fExt.md)
      |
      | F_wave =   A * cos(w * t) * Re{Fext}
      |                -  A * sin(w * t) * Im{Fext}
      |                + A * Re(Fext.md)
  Time : Inport
  Displacement : Inport  Port=2
  Add : Sum  Inputs=+++
  Add1 : Sum  Inputs=++-
  Add2 : Sum
  Constant : Constant  Value=pi/2
  Displacement Phase Enable1 : Constant  Value=body.largeXYDisplacement.option
  Excitation Imaginary Part : Constant  Value=body.hydroForce.fExt.im(1,:)  VectorParams1D=off
  Excitation Real Part : Constant  Value=body.hydroForce.fExt.re(1,:)  VectorParams1D=off
  Excitation Real Part1 : Constant  Value=body.hydroForce.fExt.md(1,:)  VectorParams1D=off
  MATLAB Function1 : MATLAB Function  TreatAsAtomicUnit=on
  Product : Product
  Product1 : Product  Inputs=3
  Product2 : Product  Inputs=3
  Product3 : Product
  Selector : Selector  IndexOptions=Index vector (dialog)  Indices=[1 2]  OutputSizes=1
  Sine Wave Function : Sin  TimeSource=Use external signal  SampleTime=0
  Sine Wave Function1 : Sin  TimeSource=Use external signal  SampleTime=0
  Wave Amplitude : Constant  Value=Nwave.amplitude(1,:)
  Wave Amplitude1 : Constant  Value=Nwave.amplitude(1,:).*Nwave.amplitude(1,:)
  Wave Frequency : Constant  Value=Nwave.omega(1,:)
  Wave Frequency1 : Constant  Value=Nwave.omega  VectorParams1D=off
  Wave Number : Constant  Value=Nwave.wavenumber
  Wave direction : Constant  Value=Nwave.direction  VectorParams1D=off
  Linear Excitation : Outport
  wires:
  Wave direction/1 -> MATLAB Function1/5(direction)
  Wave Number/1 -> MATLAB Function1/4(wavenumber)
  Wave Frequency1/1 -> MATLAB Function1/3(frequency)
  Selector/1 -> MATLAB Function1/1(disp)
  Add2/1 -> Sine Wave Function/1
  MATLAB Function1/1(dispPhase) -> Add2/2, Add/3
  Displacement Phase Enable1/1 -> MATLAB Function1/2(enable)
  Displacement/1 -> Selector/1  "t"
  Product3/1 -> Add1/1
  Excitation Real Part1/1 -> Product3/2  "Re{Fext}"
  Wave Amplitude1/1 -> Product3/1  "A"
  Constant/1 -> Add/2
  Add/1 -> Sine Wave Function1/1
  Wave Amplitude/1 -> Product1/1, Product2/1  "A"
  Add1/1 -> Linear Excitation/1
  Product2/1 -> Add1/3
  Product1/1 -> Add1/2
  Excitation Real Part/1 -> Product1/2  "Re{Fext}"
  Excitation Imaginary Part/1 -> Product2/3  "Im{Fext}"
  Sine Wave Function/1 -> Product2/2  "sin(wt)"
  Sine Wave Function1/1 -> Product1/3  "cos(w*t)"
  Product/1 -> Add/1, Add2/1
  Wave Frequency/1 -> Product/2  "w"
  Time/1 -> Product/1  "t"
